simulink model "Wind_DFIG_Average_R1"  (R2026a)
settings: Solver=ode23t  StopTime=DFIG.Simulation.StopTime  MaxStep=DFIG.Simulation.MaxStep
InitFcn:
  | root=fileparts(fileparts(get_param(bdroot,'FileName'))); run(fullfile(root,'parameters','init_wind_dfig_average_r1.m'));
undefined symbols (not defined in the file): DFIG
Description:
  | 5 MW DFIG wind turbine with explicit dq electromagnetic states and averaged rotor/grid converters. Stator is directly connected to the 690 V grid; rotor slip power flows through the shared DC link.
settings Model: Creator=fakebob2004  LastModifiedBy=fakebob2004

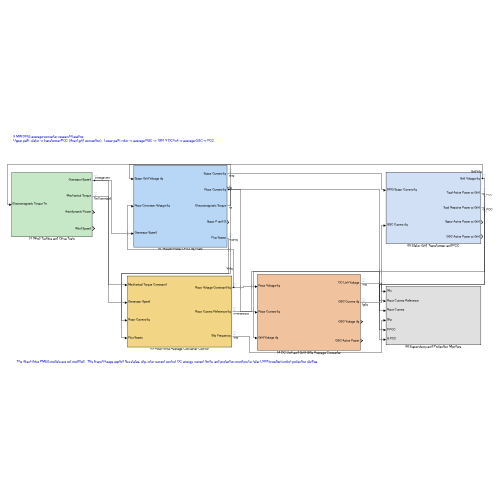
[thumbnail: Simulink's stored preview of the top-level diagram]
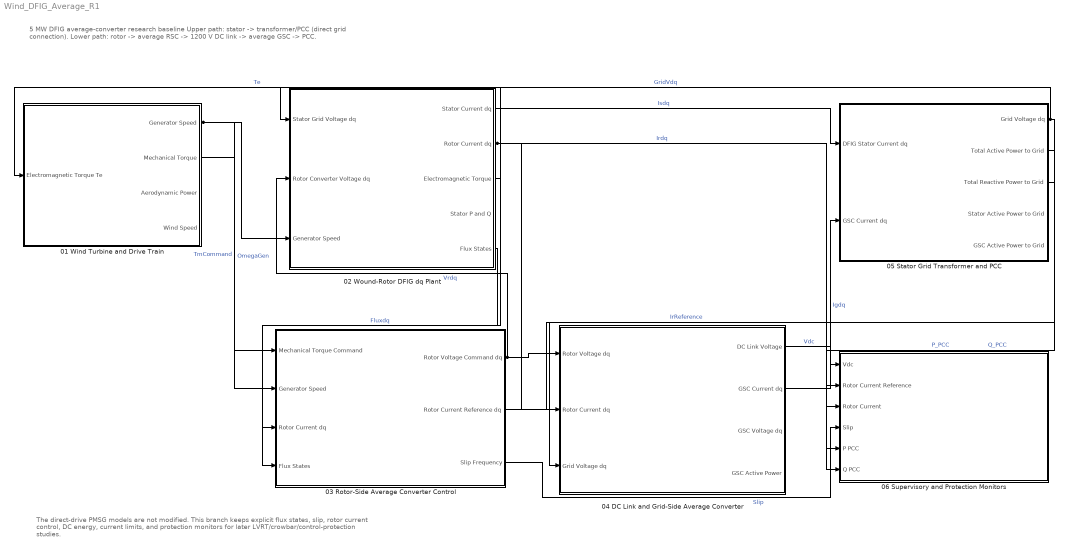
== system Wind_DFIG_Average_R1 ==
  note: 5 MW DFIG average-converter research baseline
      | Upper path: stator -> transformer/PCC (direct grid connection).  Lower path: rotor -> average RSC -> 1200 V DC link -> average GSC -> PCC.
  note: The direct-drive PMSG models are not modified. This branch keeps explicit flux states, slip, rotor current control, DC energy, current limits, and protection monitors for later LVRT/crowbar/control-protection studies.
  01 Wind Turbine and Drive Train : Subsystem
  02 Wound-Rotor DFIG dq Plant : Subsystem
  03 Rotor-Side Average Converter Control : Subsystem
  04 DC Link and Grid-Side Average Converter : Subsystem
  05 Stator Grid Transformer and PCC : Subsystem
  06 Supervisory and Protection Monitors : Subsystem
  wires:
  01 Wind Turbine and Drive Train/1(Generator Speed) -> 02 Wound-Rotor DFIG dq Plant/3(Generator Speed), 03 Rotor-Side Average Converter Control/2(Generator Speed)  "OmegaGen"
  02 Wound-Rotor DFIG dq Plant/3(Electromagnetic Torque) -> 01 Wind Turbine and Drive Train/1(Electromagnetic Torque Te)  "Te"
  01 Wind Turbine and Drive Train/2(Mechanical Torque) -> 03 Rotor-Side Average Converter Control/1(Mechanical Torque Command)  "TmCommand"
  05 Stator Grid Transformer and PCC/1(Grid Voltage dq) -> 02 Wound-Rotor DFIG dq Plant/1(Stator Grid Voltage dq), 04 DC Link and Grid-Side Average Converter/3(Grid Voltage dq)  "GridVdq"
  03 Rotor-Side Average Converter Control/1(Rotor Voltage Command dq) -> 02 Wound-Rotor DFIG dq Plant/2(Rotor Converter Voltage dq), 04 DC Link and Grid-Side Average Converter/1(Rotor Voltage dq)  "Vrdq"
  02 Wound-Rotor DFIG dq Plant/2(Rotor Current dq) -> 03 Rotor-Side Average Converter Control/3(Rotor Current dq), 04 DC Link and Grid-Side Average Converter/2(Rotor Current dq), 06 Supervisory and Protection Monitors/3(Rotor Current)  "Irdq"
  02 Wound-Rotor DFIG dq Plant/5(Flux States) -> 03 Rotor-Side Average Converter Control/4(Flux States)  "Fluxdq"
  02 Wound-Rotor DFIG dq Plant/1(Stator Current dq) -> 05 Stator Grid Transformer and PCC/1(DFIG Stator Current dq)  "Isdq"
  04 DC Link and Grid-Side Average Converter/2(GSC Current dq) -> 05 Stator Grid Transformer and PCC/2(GSC Current dq)  "Igdq"
  04 DC Link and Grid-Side Average Converter/1(DC Link Voltage) -> 06 Supervisory and Protection Monitors/1(Vdc)  "Vdc"
  03 Rotor-Side Average Converter Control/2(Rotor Current Reference dq) -> 06 Supervisory and Protection Monitors/2(Rotor Current Reference)  "IrReference"
  03 Rotor-Side Average Converter Control/3(Slip Frequency) -> 06 Supervisory and Protection Monitors/4(Slip)  "Slip"
  05 Stator Grid Transformer and PCC/2(Total Active Power to Grid) -> 06 Supervisory and Protection Monitors/5(P PCC)  "P_PCC"
  05 Stator Grid Transformer and PCC/3(Total Reactive Power to Grid) -> 06 Supervisory and Protection Monitors/6(Q PCC)  "Q_PCC"

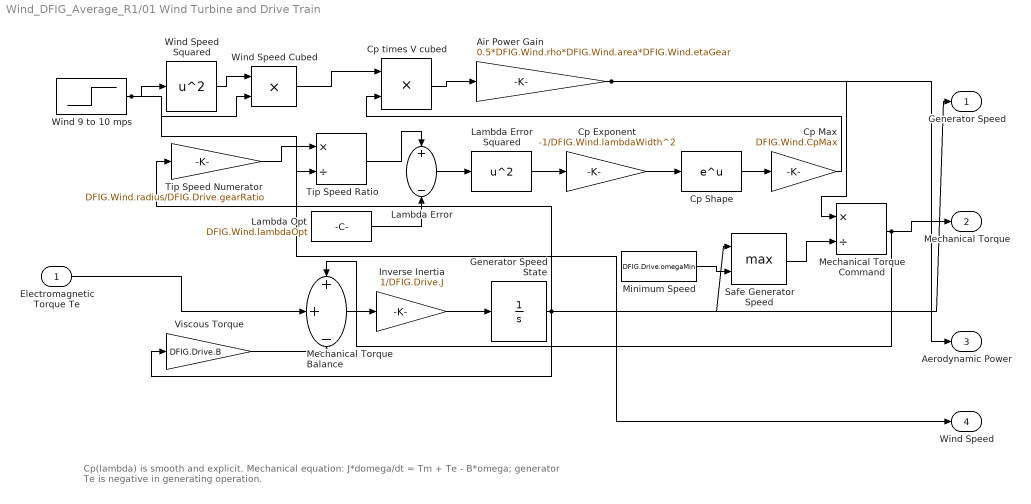
== system Wind_DFIG_Average_R1/01 Wind Turbine and Drive Train ==
  note: Cp(lambda) is smooth and explicit. Mechanical equation: J*domega/dt = Tm + Te - B*omega; generator Te is negative in generating operation.
  Electromagnetic Torque Te : Inport
  Air Power Gain : Gain  Gain=0.5*DFIG.Wind.rho*DFIG.Wind.area*DFIG.Wind.etaGear
  Cp Exponent : Gain  Gain=-1/DFIG.Wind.lambdaWidth^2
  Cp Max : Gain  Gain=DFIG.Wind.CpMax
  Cp Shape : Math
  Cp times V cubed : Product  Inputs=**
  Generator Speed State : Integrator  InitialCondition=DFIG.Drive.omega0
  Inverse Inertia : Gain  Gain=1/DFIG.Drive.J
  Lambda Error : Sum  Inputs=+-
  Lambda Error Squared : Math  Operator=square
  Lambda Opt : Constant  Value=DFIG.Wind.lambdaOpt
  Mechanical Torque Balance : Sum  Inputs=++-
  Mechanical Torque Command : Product  Inputs=*/
  Minimum Speed : Constant  Value=DFIG.Drive.omegaMin
  Safe Generator Speed : MinMax  Function=max  Inputs=2
  Tip Speed Numerator : Gain  Gain=DFIG.Wind.radius/DFIG.Drive.gearRatio
  Tip Speed Ratio : Product  Inputs=*/
  Viscous Torque : Gain  Gain=DFIG.Drive.B
  Wind 9 to 10 mps : Step  Time=DFIG.Wind.stepTime  InitialValue=DFIG.Wind.v0  FinalValue=DFIG.Wind.v0+DFIG.Wind.vStep  SampleTime=0
  Wind Speed Cubed : Product  Inputs=**
  Wind Speed Squared : Math  Operator=square
  Generator Speed : Outport
  Mechanical Torque : Outport  Port=2
  Aerodynamic Power : Outport  Port=3
  Wind Speed : Outport  Port=4
  wires:
  Wind 9 to 10 mps/1 -> Wind Speed Squared/1, Wind Speed Cubed/2, Tip Speed Ratio/2, Wind Speed/1
  Wind Speed Squared/1 -> Wind Speed Cubed/1
  Generator Speed State/1 -> Tip Speed Numerator/1, Safe Generator Speed/1, Viscous Torque/1, Generator Speed/1
  Tip Speed Numerator/1 -> Tip Speed Ratio/1
  Tip Speed Ratio/1 -> Lambda Error/1
  Lambda Opt/1 -> Lambda Error/2
  Lambda Error/1 -> Lambda Error Squared/1
  Lambda Error Squared/1 -> Cp Exponent/1
  Cp Exponent/1 -> Cp Shape/1
  Cp Shape/1 -> Cp Max/1
  Wind Speed Cubed/1 -> Cp times V cubed/1
  Cp Max/1 -> Cp times V cubed/2
  Cp times V cubed/1 -> Air Power Gain/1
  Minimum Speed/1 -> Safe Generator Speed/2
  Air Power Gain/1 -> Mechanical Torque Command/1, Aerodynamic Power/1
  Safe Generator Speed/1 -> Mechanical Torque Command/2
  Mechanical Torque Command/1 -> Mechanical Torque Balance/1, Mechanical Torque/1
  Electromagnetic Torque Te/1 -> Mechanical Torque Balance/2
  Viscous Torque/1 -> Mechanical Torque Balance/3
  Mechanical Torque Balance/1 -> Inverse Inertia/1
  Inverse Inertia/1 -> Generator Speed State/1

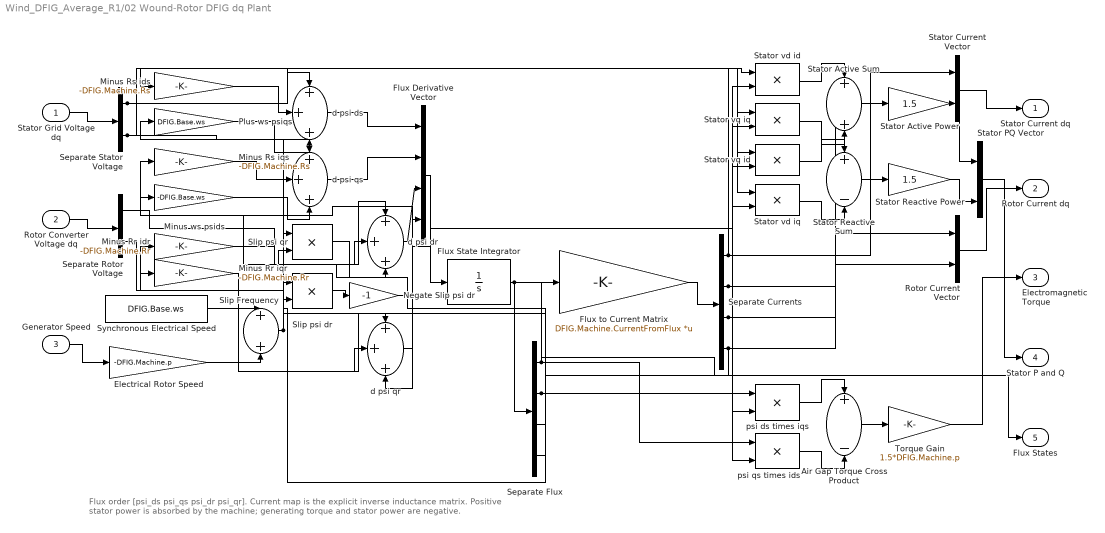
== system Wind_DFIG_Average_R1/02 Wound-Rotor DFIG dq Plant ==
  note: Flux order [psi_ds psi_qs psi_dr psi_qr]. Current map is the explicit inverse inductance matrix. Positive stator power is absorbed by the machine; generating torque and stator power are negative.
  Stator Grid Voltage dq : Inport
  Rotor Converter Voltage dq : Inport  Port=2
  Generator Speed : Inport  Port=3
  Air Gap Torque Cross Product : Sum  Inputs=+-
  Electrical Rotor Speed : Gain  Gain=-DFIG.Machine.p
  Flux Derivative Vector : Mux
  Flux State Integrator : Integrator  InitialCondition=DFIG.Initial.flux
  Flux to Current Matrix : Gain  Gain=DFIG.Machine.CurrentFromFlux  Multiplication=Matrix(K*u)
  Minus Rr idr : Gain  Gain=-DFIG.Machine.Rr
  Minus Rr iqr : Gain  Gain=-DFIG.Machine.Rr
  Minus Rs ids : Gain  Gain=-DFIG.Machine.Rs
  Minus Rs iqs : Gain  Gain=-DFIG.Machine.Rs
  Minus ws psids : Gain  Gain=-DFIG.Base.ws
  Negate Slip psi dr : Gain  Gain=-1
  Plus ws psiqs : Gain  Gain=DFIG.Base.ws
  Rotor Current Vector : Mux  Inputs=2
  Separate Currents : Demux
  Separate Flux : Demux
  Separate Rotor Voltage : Demux  Outputs=2
  Separate Stator Voltage : Demux  Outputs=2
  Slip Frequency : Sum
  Slip psi dr : Product  Inputs=**
  Slip psi qr : Product  Inputs=**
  Stator Active Power : Gain  Gain=1.5
  Stator Active Sum : Sum
  Stator Current Vector : Mux  Inputs=2
  Stator PQ Vector : Mux  Inputs=2
  Stator Reactive Power : Gain  Gain=1.5
  Stator Reactive Sum : Sum  Inputs=+-
  Stator vd id : Product  Inputs=**
  Stator vd iq : Product  Inputs=**
  Stator vq id : Product  Inputs=**
  Stator vq iq : Product  Inputs=**
  Synchronous Electrical Speed : Constant  Value=DFIG.Base.ws
  Torque Gain : Gain  Gain=1.5*DFIG.Machine.p
  d psi dr : Sum  Inputs=+++
  d psi ds : Sum  Inputs=+++
  d psi qr : Sum  Inputs=+++
  d psi qs : Sum  Inputs=+++
  psi ds times iqs : Product  Inputs=**
  psi qs times ids : Product  Inputs=**
  Stator Current dq : Outport
  Rotor Current dq : Outport  Port=2
  Electromagnetic Torque : Outport  Port=3
  Stator P and Q : Outport  Port=4
  Flux States : Outport  Port=5
  wires:
  Flux Derivative Vector/1 -> Flux State Integrator/1
  Flux State Integrator/1 -> Flux to Current Matrix/1, Separate Flux/1, Flux States/1
  Flux to Current Matrix/1 -> Separate Currents/1
  Stator Grid Voltage dq/1 -> Separate Stator Voltage/1
  Rotor Converter Voltage dq/1 -> Separate Rotor Voltage/1
  Synchronous Electrical Speed/1 -> Slip Frequency/1
  Generator Speed/1 -> Electrical Rotor Speed/1
  Electrical Rotor Speed/1 -> Slip Frequency/2
  Separate Currents/1 -> Minus Rs ids/1, psi qs times ids/2, Stator vd id/2, Stator vq id/2, Stator Current Vector/1
  Separate Flux/2 -> Plus ws psiqs/1, psi qs times ids/1
  Separate Stator Voltage/1 -> d psi ds/1, Stator vd id/1, Stator vd iq/1
  Minus Rs ids/1 -> d psi ds/2
  Plus ws psiqs/1 -> d psi ds/3
  Separate Currents/2 -> Minus Rs iqs/1, psi ds times iqs/2, Stator vq iq/2, Stator vd iq/2, Stator Current Vector/2
  Separate Flux/1 -> Minus ws psids/1, psi ds times iqs/1
  Separate Stator Voltage/2 -> d psi qs/1, Stator vq iq/1, Stator vq id/1
  Minus Rs iqs/1 -> d psi qs/2
  Minus ws psids/1 -> d psi qs/3
  Separate Currents/3 -> Minus Rr idr/1, Rotor Current Vector/1
  Slip Frequency/1 -> Slip psi qr/1, Slip psi dr/1
  Separate Flux/4 -> Slip psi qr/2
  Separate Rotor Voltage/1 -> d psi dr/1
  Minus Rr idr/1 -> d psi dr/2
  Slip psi qr/1 -> d psi dr/3
  Separate Currents/4 -> Minus Rr iqr/1, Rotor Current Vector/2
  Separate Flux/3 -> Slip psi dr/2
  Slip psi dr/1 -> Negate Slip psi dr/1
  Separate Rotor Voltage/2 -> d psi qr/1
  Minus Rr iqr/1 -> d psi qr/2
  Negate Slip psi dr/1 -> d psi qr/3
  d psi ds/1 -> Flux Derivative Vector/1
  d psi qs/1 -> Flux Derivative Vector/2
  d psi dr/1 -> Flux Derivative Vector/3
  d psi qr/1 -> Flux Derivative Vector/4
  psi ds times iqs/1 -> Air Gap Torque Cross Product/1
  psi qs times ids/1 -> Air Gap Torque Cross Product/2
  Air Gap Torque Cross Product/1 -> Torque Gain/1
  Stator vd id/1 -> Stator Active Sum/1
  Stator vq iq/1 -> Stator Active Sum/2
  Stator Active Sum/1 -> Stator Active Power/1
  Stator vq id/1 -> Stator Reactive Sum/1
  Stator vd iq/1 -> Stator Reactive Sum/2
  Stator Reactive Sum/1 -> Stator Reactive Power/1
  Stator Active Power/1 -> Stator PQ Vector/1
  Stator Reactive Power/1 -> Stator PQ Vector/2
  Stator Current Vector/1 -> Stator Current dq/1
  Rotor Current Vector/1 -> Rotor Current dq/1
  Torque Gain/1 -> Electromagnetic Torque/1
  Stator PQ Vector/1 -> Stator P and Q/1

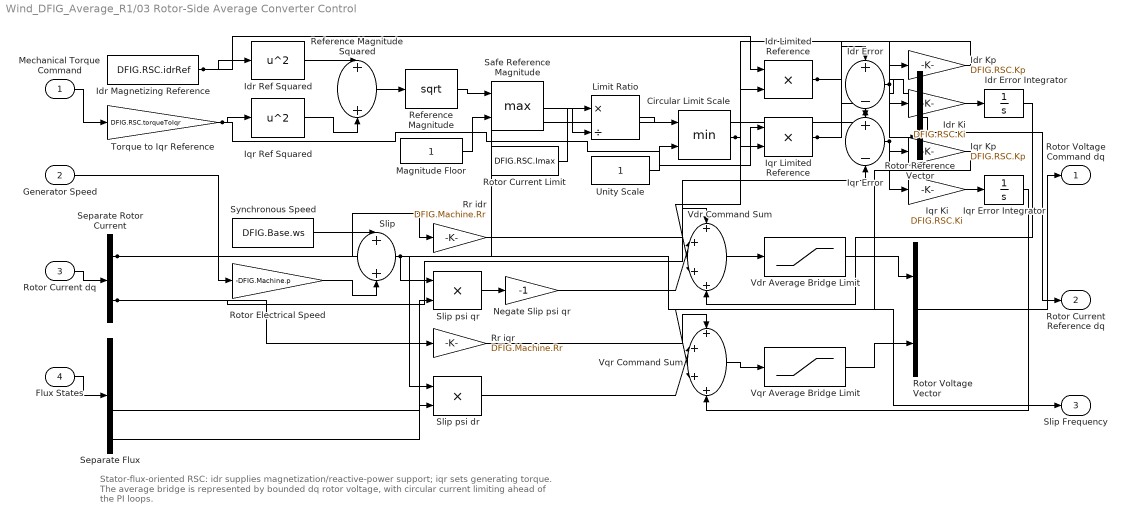
== system Wind_DFIG_Average_R1/03 Rotor-Side Average Converter Control ==
  note: Stator-flux-oriented RSC: idr supplies magnetization/reactive-power support; iqr sets generating torque. The average bridge is represented by bounded dq rotor voltage, with circular current limiting ahead of the PI loops.
  Mechanical Torque Command : Inport
  Generator Speed : Inport  Port=2
  Rotor Current dq : Inport  Port=3
  Flux States : Inport  Port=4
  Circular Limit Scale : MinMax  Inputs=2
  Idr Error : Sum  Inputs=+-
  Idr Error Integrator : Integrator
  Idr Ki : Gain  Gain=DFIG.RSC.Ki
  Idr Kp : Gain  Gain=DFIG.RSC.Kp
  Idr Limited Reference : Product  Inputs=**
  Idr Magnetizing Reference : Constant  Value=DFIG.RSC.idrRef
  Idr Ref Squared : Math  Operator=square
  Iqr Error : Sum  Inputs=+-
  Iqr Error Integrator : Integrator
  Iqr Ki : Gain  Gain=DFIG.RSC.Ki
  Iqr Kp : Gain  Gain=DFIG.RSC.Kp
  Iqr Limited Reference : Product  Inputs=**
  Iqr Ref Squared : Math  Operator=square
  Limit Ratio : Product  Inputs=*/
  Magnitude Floor : Constant
  Negate Slip psi qr : Gain  Gain=-1
  Reference Magnitude : Math  Operator=sqrt
  Reference Magnitude Squared : Sum
  Rotor Current Limit : Constant  Value=DFIG.RSC.Imax
  Rotor Electrical Speed : Gain  Gain=-DFIG.Machine.p
  Rotor Reference Vector : Mux  Inputs=2
  Rotor Voltage Vector : Mux  Inputs=2
  Rr idr : Gain  Gain=DFIG.Machine.Rr
  Rr iqr : Gain  Gain=DFIG.Machine.Rr
  Safe Reference Magnitude : MinMax  Function=max  Inputs=2
  Separate Flux : Demux
  Separate Rotor Current : Demux  Outputs=2
  Slip : Sum
  Slip psi dr : Product  Inputs=**
  Slip psi qr : Product  Inputs=**
  Synchronous Speed : Constant  Value=DFIG.Base.ws
  Torque to Iqr Reference : Gain  Gain=DFIG.RSC.torqueToIqr
  Unity Scale : Constant
  Vdr Average Bridge Limit : Saturate  UpperLimit=DFIG.RSC.Vmax  LowerLimit=-DFIG.RSC.Vmax
  Vdr Command Sum : Sum  Inputs=++++
  Vqr Average Bridge Limit : Saturate  UpperLimit=DFIG.RSC.Vmax  LowerLimit=-DFIG.RSC.Vmax
  Vqr Command Sum : Sum  Inputs=++++
  Rotor Voltage Command dq : Outport
  Rotor Current Reference dq : Outport  Port=2
  Slip Frequency : Outport  Port=3
  wires:
  Mechanical Torque Command/1 -> Torque to Iqr Reference/1
  Idr Magnetizing Reference/1 -> Idr Ref Squared/1, Idr Limited Reference/1
  Torque to Iqr Reference/1 -> Iqr Ref Squared/1, Iqr Limited Reference/1
  Idr Ref Squared/1 -> Reference Magnitude Squared/1
  Iqr Ref Squared/1 -> Reference Magnitude Squared/2
  Reference Magnitude Squared/1 -> Reference Magnitude/1
  Reference Magnitude/1 -> Safe Reference Magnitude/1
  Magnitude Floor/1 -> Safe Reference Magnitude/2
  Rotor Current Limit/1 -> Limit Ratio/1
  Safe Reference Magnitude/1 -> Limit Ratio/2
  Limit Ratio/1 -> Circular Limit Scale/1
  Unity Scale/1 -> Circular Limit Scale/2
  Circular Limit Scale/1 -> Idr Limited Reference/2, Iqr Limited Reference/2
  Rotor Current dq/1 -> Separate Rotor Current/1
  Flux States/1 -> Separate Flux/1
  Idr Limited Reference/1 -> Idr Error/1, Rotor Reference Vector/1
  Separate Rotor Current/1 -> Idr Error/2, Rr idr/1
  Iqr Limited Reference/1 -> Iqr Error/1, Rotor Reference Vector/2
  Separate Rotor Current/2 -> Iqr Error/2, Rr iqr/1
  Idr Error/1 -> Idr Kp/1, Idr Ki/1
  Idr Ki/1 -> Idr Error Integrator/1
  Iqr Error/1 -> Iqr Kp/1, Iqr Ki/1
  Iqr Ki/1 -> Iqr Error Integrator/1
  Synchronous Speed/1 -> Slip/1
  Generator Speed/1 -> Rotor Electrical Speed/1
  Rotor Electrical Speed/1 -> Slip/2
  Slip/1 -> Slip psi qr/1, Slip psi dr/1, Slip Frequency/1
  Separate Flux/4 -> Slip psi qr/2
  Slip psi qr/1 -> Negate Slip psi qr/1
  Separate Flux/3 -> Slip psi dr/2
  Rr idr/1 -> Vdr Command Sum/1
  Negate Slip psi qr/1 -> Vdr Command Sum/2
  Idr Kp/1 -> Vdr Command Sum/3
  Idr Error Integrator/1 -> Vdr Command Sum/4
  Rr iqr/1 -> Vqr Command Sum/1
  Slip psi dr/1 -> Vqr Command Sum/2
  Iqr Kp/1 -> Vqr Command Sum/3
  Iqr Error Integrator/1 -> Vqr Command Sum/4
  Vdr Command Sum/1 -> Vdr Average Bridge Limit/1
  Vqr Command Sum/1 -> Vqr Average Bridge Limit/1
  Vdr Average Bridge Limit/1 -> Rotor Voltage Vector/1
  Vqr Average Bridge Limit/1 -> Rotor Voltage Vector/2
  Rotor Voltage Vector/1 -> Rotor Voltage Command dq/1
  Rotor Reference Vector/1 -> Rotor Current Reference dq/1

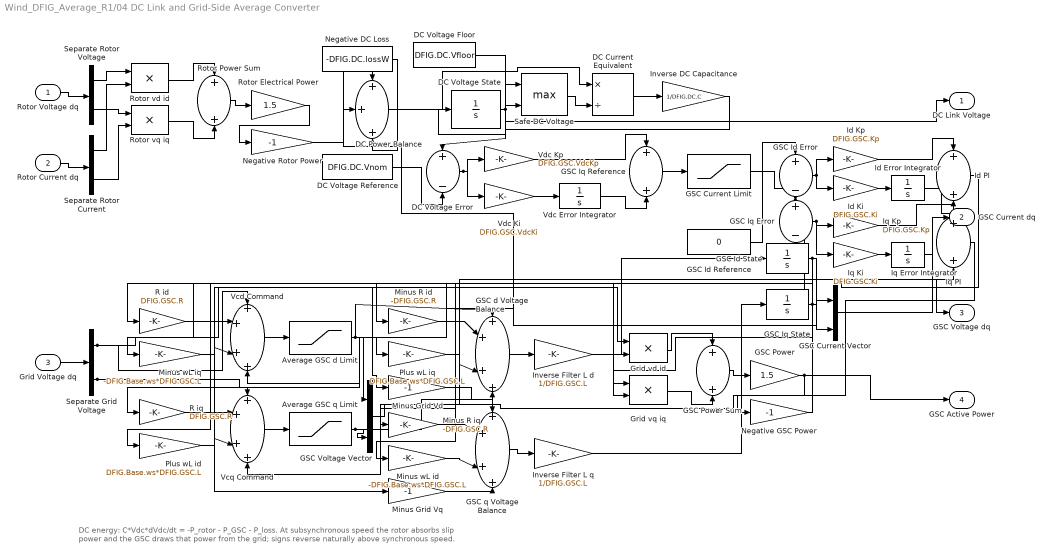
== system Wind_DFIG_Average_R1/04 DC Link and Grid-Side Average Converter ==
  note: DC energy: C*Vdc*dVdc/dt = -P_rotor - P_GSC - P_loss. At subsynchronous speed the rotor absorbs slip power and the GSC draws that power from the grid; signs reverse naturally above synchronous speed.
  Rotor Voltage dq : Inport
  Rotor Current dq : Inport  Port=2
  Grid Voltage dq : Inport  Port=3
  Average GSC d Limit : Saturate  UpperLimit=DFIG.GSC.Vmax  LowerLimit=-DFIG.GSC.Vmax
  Average GSC q Limit : Saturate  UpperLimit=DFIG.GSC.Vmax  LowerLimit=-DFIG.GSC.Vmax
  DC Current Equivalent : Product  Inputs=*/
  DC Power Balance : Sum  Inputs=+++
  DC Voltage Error : Sum  Inputs=+-
  DC Voltage Floor : Constant  Value=DFIG.DC.Vfloor
  DC Voltage Reference : Constant  Value=DFIG.DC.Vnom
  DC Voltage State : Integrator  InitialCondition=DFIG.DC.Vnom
  GSC Current Limit : Saturate  UpperLimit=DFIG.GSC.Imax  LowerLimit=-DFIG.GSC.Imax
  GSC Current Vector : Mux  Inputs=2
  GSC Id Error : Sum  Inputs=+-
  GSC Id Reference : Constant  Value=0
  GSC Id State : Integrator
  GSC Iq Error : Sum  Inputs=+-
  GSC Iq Reference : Sum
  GSC Iq State : Integrator  InitialCondition=DFIG.Initial.igqGSC
  GSC Power : Gain  Gain=1.5
  GSC Power Sum : Sum
  GSC Voltage Vector : Mux  Inputs=2
  GSC d Voltage Balance : Sum  Inputs=++++
  GSC q Voltage Balance : Sum  Inputs=++++
  Grid vd id : Product  Inputs=**
  Grid vq iq : Product  Inputs=**
  Id Error Integrator : Integrator
  Id Ki : Gain  Gain=DFIG.GSC.Ki
  Id Kp : Gain  Gain=DFIG.GSC.Kp
  Id PI : Sum
  Inverse DC Capacitance : Gain  Gain=1/DFIG.DC.C
  Inverse Filter L d : Gain  Gain=1/DFIG.GSC.L
  Inverse Filter L q : Gain  Gain=1/DFIG.GSC.L
  Iq Error Integrator : Integrator
  Iq Ki : Gain  Gain=DFIG.GSC.Ki
  Iq Kp : Gain  Gain=DFIG.GSC.Kp
  Iq PI : Sum
  Minus Grid Vd : Gain  Gain=-1
  Minus Grid Vq : Gain  Gain=-1
  Minus R id : Gain  Gain=-DFIG.GSC.R
  Minus R iq : Gain  Gain=-DFIG.GSC.R
  Minus wL id : Gain  Gain=-DFIG.Base.ws*DFIG.GSC.L
  Minus wL iq : Gain  Gain=-DFIG.Base.ws*DFIG.GSC.L
  Negative DC Loss : Constant  Value=-DFIG.DC.lossW
  Negative GSC Power : Gain  Gain=-1
  Negative Rotor Power : Gain  Gain=-1
  Plus wL id : Gain  Gain=DFIG.Base.ws*DFIG.GSC.L
  Plus wL iq : Gain  Gain=DFIG.Base.ws*DFIG.GSC.L
  R id : Gain  Gain=DFIG.GSC.R
  R iq : Gain  Gain=DFIG.GSC.R
  Rotor Electrical Power : Gain  Gain=1.5
  Rotor Power Sum : Sum
  Rotor vd id : Product  Inputs=**
  Rotor vq iq : Product  Inputs=**
  Safe DC Voltage : MinMax  Function=max  Inputs=2
  Separate Grid Voltage : Demux  Outputs=2
  Separate Rotor Current : Demux  Outputs=2
  Separate Rotor Voltage : Demux  Outputs=2
  Vcd Command : Sum  Inputs=++++
  Vcq Command : Sum  Inputs=++++
  Vdc Error Integrator : Integrator  InitialCondition=DFIG.Initial.igqGSC
  Vdc Ki : Gain  Gain=DFIG.GSC.VdcKi
  Vdc Kp : Gain  Gain=DFIG.GSC.VdcKp
  DC Link Voltage : Outport
  GSC Current dq : Outport  Port=2
  GSC Voltage dq : Outport  Port=3
  GSC Active Power : Outport  Port=4
  wires:
  Rotor Voltage dq/1 -> Separate Rotor Voltage/1
  Rotor Current dq/1 -> Separate Rotor Current/1
  Separate Rotor Voltage/1 -> Rotor vd id/1
  Separate Rotor Current/1 -> Rotor vd id/2
  Separate Rotor Voltage/2 -> Rotor vq iq/1
  Separate Rotor Current/2 -> Rotor vq iq/2
  Rotor vd id/1 -> Rotor Power Sum/1
  Rotor vq iq/1 -> Rotor Power Sum/2
  Rotor Power Sum/1 -> Rotor Electrical Power/1
  DC Voltage State/1 -> DC Voltage Error/1, Safe DC Voltage/1, DC Link Voltage/1
  DC Voltage Reference/1 -> DC Voltage Error/2
  DC Voltage Error/1 -> Vdc Kp/1, Vdc Ki/1
  Vdc Ki/1 -> Vdc Error Integrator/1
  Vdc Kp/1 -> GSC Iq Reference/1
  Vdc Error Integrator/1 -> GSC Iq Reference/2
  GSC Iq Reference/1 -> GSC Current Limit/1
  Grid Voltage dq/1 -> Separate Grid Voltage/1
  GSC Id Reference/1 -> GSC Id Error/1
  GSC Id State/1 -> GSC Id Error/2, R id/1, Plus wL id/1, Minus R id/1, Minus wL id/1, Grid vd id/2, GSC Current Vector/1
  GSC Current Limit/1 -> GSC Iq Error/1
  GSC Iq State/1 -> GSC Iq Error/2, Minus wL iq/1, R iq/1, Plus wL iq/1, Minus R iq/1, Grid vq iq/2, GSC Current Vector/2
  GSC Id Error/1 -> Id Kp/1, Id Ki/1
  Id Ki/1 -> Id Error Integrator/1
  Id Kp/1 -> Id PI/1
  Id Error Integrator/1 -> Id PI/2
  GSC Iq Error/1 -> Iq Kp/1, Iq Ki/1
  Iq Ki/1 -> Iq Error Integrator/1
  Iq Kp/1 -> Iq PI/1
  Iq Error Integrator/1 -> Iq PI/2
  Separate Grid Voltage/1 -> Vcd Command/1, Minus Grid Vd/1, Grid vd id/1
  R id/1 -> Vcd Command/2
  Minus wL iq/1 -> Vcd Command/3
  Id PI/1 -> Vcd Command/4
  Vcd Command/1 -> Average GSC d Limit/1
  Separate Grid Voltage/2 -> Vcq Command/1, Minus Grid Vq/1, Grid vq iq/1
  R iq/1 -> Vcq Command/2
  Plus wL id/1 -> Vcq Command/3
  Iq PI/1 -> Vcq Command/4
  Vcq Command/1 -> Average GSC q Limit/1
  Average GSC d Limit/1 -> GSC d Voltage Balance/1, GSC Voltage Vector/1
  Minus R id/1 -> GSC d Voltage Balance/2
  Plus wL iq/1 -> GSC d Voltage Balance/3
  Minus Grid Vd/1 -> GSC d Voltage Balance/4
  GSC d Voltage Balance/1 -> Inverse Filter L d/1
  Inverse Filter L d/1 -> GSC Id State/1
  Average GSC q Limit/1 -> GSC q Voltage Balance/1, GSC Voltage Vector/2
  Minus R iq/1 -> GSC q Voltage Balance/2
  Minus wL id/1 -> GSC q Voltage Balance/3
  Minus Grid Vq/1 -> GSC q Voltage Balance/4
  GSC q Voltage Balance/1 -> Inverse Filter L q/1
  Inverse Filter L q/1 -> GSC Iq State/1
  Grid vd id/1 -> GSC Power Sum/1
  Grid vq iq/1 -> GSC Power Sum/2
  GSC Power Sum/1 -> GSC Power/1
  Rotor Electrical Power/1 -> Negative Rotor Power/1
  GSC Power/1 -> Negative GSC Power/1, GSC Active Power/1
  Negative Rotor Power/1 -> DC Power Balance/1
  Negative GSC Power/1 -> DC Power Balance/2
  Negative DC Loss/1 -> DC Power Balance/3
  DC Voltage Floor/1 -> Safe DC Voltage/2
  DC Power Balance/1 -> DC Current Equivalent/1
  Safe DC Voltage/1 -> DC Current Equivalent/2
  DC Current Equivalent/1 -> Inverse DC Capacitance/1
  Inverse DC Capacitance/1 -> DC Voltage State/1
  GSC Current Vector/1 -> GSC Current dq/1
  GSC Voltage Vector/1 -> GSC Voltage dq/1

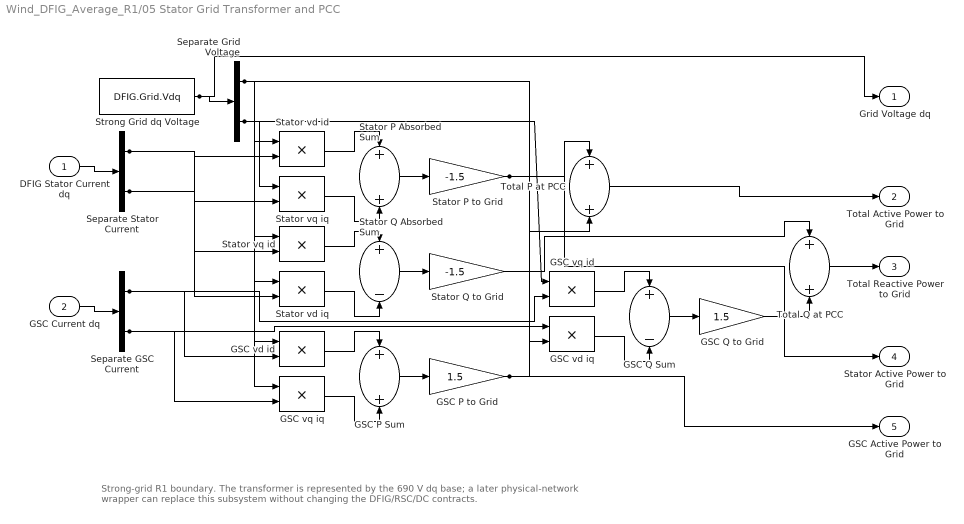
== system Wind_DFIG_Average_R1/05 Stator Grid Transformer and PCC ==
  note: Strong-grid R1 boundary. The transformer is represented by the 690 V dq base; a later physical-network wrapper can replace this subsystem without changing the DFIG/RSC/DC contracts.
  DFIG Stator Current dq : Inport
  GSC Current dq : Inport  Port=2
  GSC P Sum : Sum
  GSC P to Grid : Gain  Gain=1.5
  GSC Q Sum : Sum  Inputs=+-
  GSC Q to Grid : Gain  Gain=1.5
  GSC vd id : Product  Inputs=**
  GSC vd iq : Product  Inputs=**
  GSC vq id : Product  Inputs=**
  GSC vq iq : Product  Inputs=**
  Separate GSC Current : Demux  Outputs=2
  Separate Grid Voltage : Demux  Outputs=2
  Separate Stator Current : Demux  Outputs=2
  Stator P Absorbed Sum : Sum
  Stator P to Grid : Gain  Gain=-1.5
  Stator Q Absorbed Sum : Sum  Inputs=+-
  Stator Q to Grid : Gain  Gain=-1.5
  Stator vd id : Product  Inputs=**
  Stator vd iq : Product  Inputs=**
  Stator vq id : Product  Inputs=**
  Stator vq iq : Product  Inputs=**
  Strong Grid dq Voltage : Constant  Value=DFIG.Grid.Vdq
  Total P at PCC : Sum
  Total Q at PCC : Sum
  Grid Voltage dq : Outport
  Total Active Power to Grid : Outport  Port=2
  Total Reactive Power to Grid : Outport  Port=3
  Stator Active Power to Grid : Outport  Port=4
  GSC Active Power to Grid : Outport  Port=5
  wires:
  Strong Grid dq Voltage/1 -> Separate Grid Voltage/1, Grid Voltage dq/1
  DFIG Stator Current dq/1 -> Separate Stator Current/1
  GSC Current dq/1 -> Separate GSC Current/1
  Separate Grid Voltage/1 -> Stator vd id/1, Stator vd iq/1, GSC vd id/1, GSC vd iq/1
  Separate Stator Current/1 -> Stator vd id/2, Stator vq id/2
  Separate Grid Voltage/2 -> Stator vq iq/1, Stator vq id/1, GSC vq iq/1, GSC vq id/1
  Separate Stator Current/2 -> Stator vq iq/2, Stator vd iq/2
  Stator vd id/1 -> Stator P Absorbed Sum/1
  Stator vq iq/1 -> Stator P Absorbed Sum/2
  Stator P Absorbed Sum/1 -> Stator P to Grid/1
  Stator vq id/1 -> Stator Q Absorbed Sum/1
  Stator vd iq/1 -> Stator Q Absorbed Sum/2
  Stator Q Absorbed Sum/1 -> Stator Q to Grid/1
  Separate GSC Current/1 -> GSC vd id/2, GSC vq id/2
  Separate GSC Current/2 -> GSC vq iq/2, GSC vd iq/2
  GSC vd id/1 -> GSC P Sum/1
  GSC vq iq/1 -> GSC P Sum/2
  GSC P Sum/1 -> GSC P to Grid/1
  GSC vq id/1 -> GSC Q Sum/1
  GSC vd iq/1 -> GSC Q Sum/2
  GSC Q Sum/1 -> GSC Q to Grid/1
  Stator P to Grid/1 -> Total P at PCC/1, Stator Active Power to Grid/1
  GSC P to Grid/1 -> Total P at PCC/2, GSC Active Power to Grid/1
  Stator Q to Grid/1 -> Total Q at PCC/1
  GSC Q to Grid/1 -> Total Q at PCC/2
  Total P at PCC/1 -> Total Active Power to Grid/1
  Total Q at PCC/1 -> Total Reactive Power to Grid/1

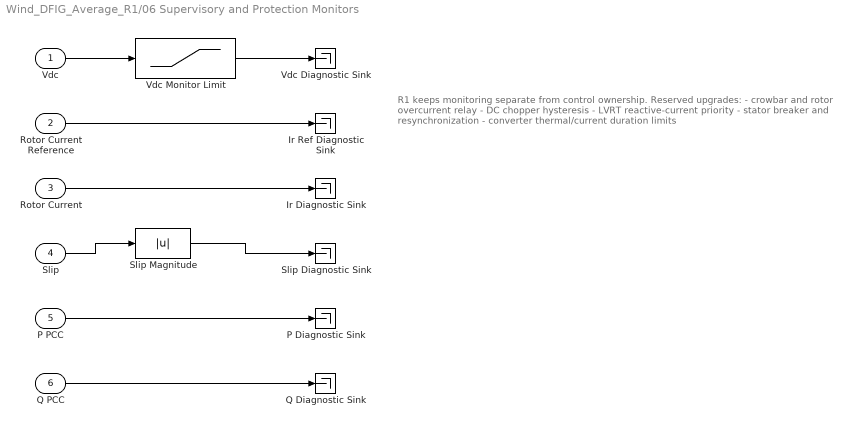
== system Wind_DFIG_Average_R1/06 Supervisory and Protection Monitors ==
  note: R1 keeps monitoring separate from control ownership.\n\nReserved upgrades:\n - crowbar and rotor overcurrent relay\n - DC chopper hysteresis\n - LVRT reactive-current priority\n - stator breaker and resynchronization\n - converter thermal/current duration limits
  Vdc : Inport
  Rotor Current Reference : Inport  Port=2
  Rotor Current : Inport  Port=3
  Slip : Inport  Port=4
  P PCC : Inport  Port=5
  Q PCC : Inport  Port=6
  Ir Diagnostic Sink : Terminator
  Ir Ref Diagnostic Sink : Terminator
  P Diagnostic Sink : Terminator
  Q Diagnostic Sink : Terminator
  Slip Diagnostic Sink : Terminator
  Slip Magnitude : Abs  SaturateOnIntegerOverflow=off
  Vdc Diagnostic Sink : Terminator
  Vdc Monitor Limit : Saturate  UpperLimit=1.20*DFIG.DC.Vnom  LowerLimit=0.80*DFIG.DC.Vnom
  wires:
  Vdc/1 -> Vdc Monitor Limit/1
  Vdc Monitor Limit/1 -> Vdc Diagnostic Sink/1
  Rotor Current Reference/1 -> Ir Ref Diagnostic Sink/1
  Rotor Current/1 -> Ir Diagnostic Sink/1
  Slip/1 -> Slip Magnitude/1
  Slip Magnitude/1 -> Slip Diagnostic Sink/1
  P PCC/1 -> P Diagnostic Sink/1
  Q PCC/1 -> Q Diagnostic Sink/1
